simulink model "text_6"  (R2022a)
settings: Solver=VariableStepAuto  StartTime=0.0  StopTime=10.0  RelTol=1e-3
libraries: dsparch4 x1
settings Model: Creator=刘笑  LastModifiedBy=刘笑

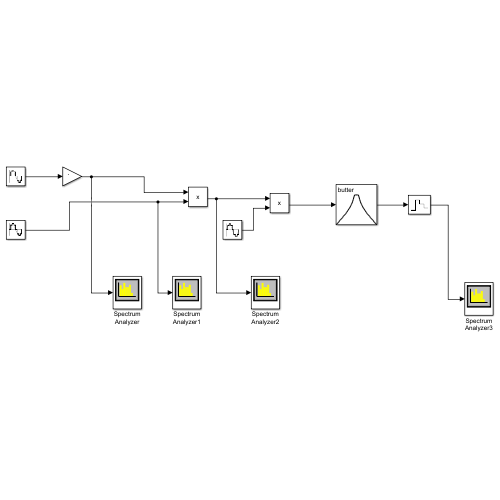
[thumbnail: Simulink's stored preview of the top-level diagram]
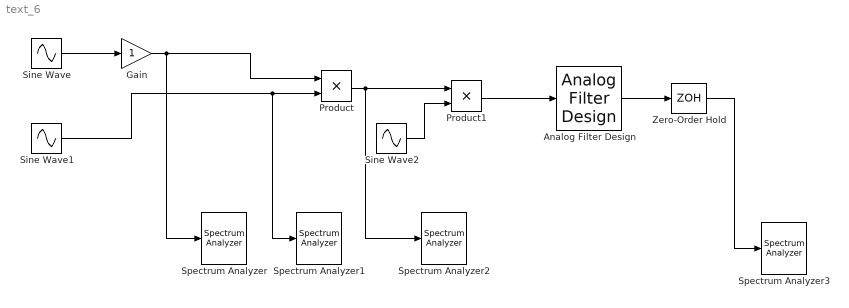
== system text_6 ==
  Analog Filter Design : dsparch4/Analog Filter Design  method=Butterworth  filttype=Bandpass  N=8  Wlo=80*2*pi  Whi=120*2*pi  Rp=2  Rs=40
  Gain : Gain
  Product : Product
  Product1 : Product
  Sine Wave : Sin  Frequency=100*2*pi  SampleTime=0.001
  Sine Wave1 : Sin  Frequency=140*2*pi  SampleTime=0.001
  Sine Wave2 : Sin  Frequency=140*2*pi  SampleTime=0.001
  Spectrum Analyzer{,1..3} (4 alike) : SpectrumAnalyzer
  Zero-Order Hold : ZeroOrderHold  SampleTime=0.001
  wires:
  Sine Wave/1 -> Gain/1
  Gain/1 -> Spectrum Analyzer/1, Product/1
  Sine Wave1/1 -> Spectrum Analyzer1/1, Product/2
  Product/1 -> Spectrum Analyzer2/1, Product1/1
  Sine Wave2/1 -> Product1/2
  Product1/1 -> Analog Filter Design/1
  Analog Filter Design/1 -> Zero-Order Hold/1
  Zero-Order Hold/1 -> Spectrum Analyzer3/1
